simulink model "grid_afe_n"  (R2026a)
settings: Solver=ode23tb  StopTime=simlength  FixedStep=tc  MaxStep=glb_time.tc
values from neighbouring files (symbols this model uses):
  afe_ctrl = ctrl_afe_setup(glb_time.ts_afe, grid_emu.omega_grid_nom)    [init_model.m]
  afe_pwm_phase_shift_mod1 = 0    [init_model.m]
  afe_pwm_phase_shift_mod2 = 0    [init_model.m]
  afe_pwm_phase_shift_mod3 = 0    [init_model.m]
  afe_pwm_phase_shift_mod4 = 0    [init_model.m]
  filters = setup_global_filters(glb_time.ts_afe, glb_time.ts_inv, glb_time.ts_dab, glb_time.tc)    [init_model.m]
  frt_data = frt_settings(test_index, test_subindex, asymmetric_error_type,      enable_frt_1, enable_frt_2, start_time_LVRT, deepPOSxi, deepPOSeta, deepNEGxi, deepNEGeta)    [init_model.m]
  glb_time = timing_setup(fpwm_afe, trgo_afe, fpwm_inv, trgo_inv, fpwm_single_phase_inv, trgo_single_phase_inv, fpwm_dab, trgo_dab,      fpwm_psfbc, trgo_psfbc, fpwm_isop_rail, trgo_isop_rail, fpwm_cllc, trgo_cllc, t_measure, tc_factor, tc_decimation, delay_pwm, dead_time_afe,      dead_time_inv, dead_time_single_phase_inv, dead_time_dab, dead_time_psfbc, dead_time_isop_rail, dead_time_cllc)    [init_model.m]
  grid_emu = grid_three_phase_emulator('Dyn11', delta_star, grid_nominal_power, application_voltage, us1, us2, fgrid,                  eq_grid_inductance, eq_grid_resistance, eta, ucc, i1m, p_iron, n1, n2, core_area, core_length, mur,                  up_xi_pu_ref, up_eta_pu_ref, un_xi_pu_ref, un_eta_pu_ref)    [init_model.m]
  i_react_pos_ref_2 = -ixi_ref_mod1*tan(acos(0.95))    [init_model.m]
  i_react_pos_ref_3 = ixi_ref_mod1*tan(acos(0.95))    [init_model.m]
  ixi_ref_mod1 = -0.85    [init_model.m]
  ixi_ref_mod2 = -0.85    [init_model.m]
  ixi_ref_mod3 = -0.85    [init_model.m]
  ixi_ref_mod4 = -0.85    [init_model.m]
  ki_align = 18    [init_model.m]
  kp_align = 0.25    [init_model.m]
  lim_down_align = -0.05    [init_model.m]
  lim_up_align = 0.05    [init_model.m]
  mavarage_filter_frequency_base_order = 2    [init_model.m]
  time_gain_afe_module_1 = 1.0002    [init_model.m]
  time_gain_afe_module_2 = 1.0015    [init_model.m]
  time_gain_afe_module_3 = 0.9988    [init_model.m]
  time_gain_afe_module_4 = 1.0020    (= 1.002)    [init_model.m]
  time_i_react_pos_ref_1 = start_time_LVRT + error_length + 0.335    [init_model.m]
  time_i_react_pos_ref_2 = time_i_react_pos_ref_1 + 0.5    (= 0.5)    [init_model.m]
  u_cm_comp_mod1 = 0    [init_model.m]
  u_cm_comp_mod2 = -1    [init_model.m]
  u_cm_comp_mod3 = -1    [init_model.m]
  u_cm_comp_mod4 = -1    [init_model.m]
undefined symbols (not defined in the file or in its folder): hwdata, magnitude
libraries: fl_lib x113, nesl_utility x75, moving_average_filter x40, moving_average_filter_cc x32, sl_discontinuities x12, linear_double_integrator_observer_ccaller x8, discrete_time_low_pass_filter x4, threephase_inductor_lib x4, dclink_for_two_levels x4, three_phase_pwm_modulator x4, three_phase_inverter_ideal_switch_based_model x4, three_phase_inverter_igbt_advanced_thermal_model x4
(part 11 of 19)

== system grid_afe_n/afe_abc_mod1/AFE_control/afe_control/grid_voltage_phase_lock_loops/dq_pll/pll_stageB ==
  u_grid_pos_xi : Inport
  u_grid_pos_eta : Inport  Port=2
  -2<x<2 : Saturate  UpperLimit=2  LowerLimit=-2
  Constant4 : Constant  Value=grid_emu.omega_grid_nom
  Gain : Gain  Gain=1/grid_emu.omega_grid_nom
  Product1 : Product  RndMeth=Zero
  Product2 : Product  RndMeth=Zero
  Sum3 : Sum  SaturateOnIntegerOverflow=on
  Sum4 : Sum  SaturateOnIntegerOverflow=on
  Sum5 : Sum  Inputs=++|
  Terminator : Terminator
  Unit Delay1 : UnitDelay  SampleTime=-1
  Unit Delay2 : UnitDelay  SampleTime=-1
  Unit Delay4 : UnitDelay  SampleTime=-1
  bounder1 : MATLAB Function  TreatAsAtomicUnit=on
  double_integrator_observer : Subsystem
  kp : Gain  Gain=afe_ctrl.pll_i1*glb_time.ts_afe  SaturateOnIntegerOverflow=on  OutDataTypeStr=Inherit: Same as input  ParamDataTypeStr=Inherit: Same as input
  kp2 : Gain  Gain=glb_time.ts_afe  SaturateOnIntegerOverflow=on  OutDataTypeStr=Inherit: Same as input  ParamDataTypeStr=Inherit: Same as input
  scheduled-p-gain : Subsystem
      settings: PortSchema="{\"entries\":[{\"content\":{\"sides\":[{\"content\":{},\"type\":\"ConnectorPlacement.EquallySpacedRectSide\",\"uuid\":\"88e64df2-a299-4c1b-9bac-7a615cd04a00\"},{\"content\":{\"side\":\"RIGHT\"},\"type\":\"ConnectorPlacement.EquallySpacedRectSide\",\"uuid\":\"ef1d7318-b0e2-4e96-bf99-c42bb4ec5202\"},{\"content\":{\"connectorIds\":[\"In1\"],\"side\":\"TOP\"},\"type\":\"ConnectorPlacement.EquallySpacedRectSide\",\"uuid\":\"96582c59-f6c8-40f1-b3cf-394cc239c4b2\"},{\"content\":{\"connectorIds\":[\"Out1\"],\"side\":\"BOTTOM\"},\"type\":\"ConnectorPlacement.EquallySpacedRectSide\",\"uuid\":\"9ac5cd0d-958f-4b67-b4ea-90856a0aa038\"}]},\"type\":\"ConnectorPlacement.EquallySpacedConnector\",\"uuid\":\"ca37db80-6b94-4315-bd9c-66307567cd1f\"}],\"packageUris\":[\"http://schema.mathworks.com/mf0/Connector/R2020b\"],\"version\":\"1.0\"}"
  phase_grid_pll : Outport  VectorParamsAs1DForOutWhenUnconnected=off
  omega_grid_pu_pll : Outport  Port=2  VectorParamsAs1DForOutWhenUnconnected=off
  wires:
  Unit Delay4/1 -> Sum3/2
  Sum3/1 -> -2<x<2/1
  Sum4/1 -> bounder1/1(u)
  Unit Delay1/1 -> Sum4/2
  -2<x<2/1 -> Sum5/2, Unit Delay4/1  "i1"
  kp2/1 -> Sum4/1
  Constant4/1 -> Product2/2
  [Vgrid_unorm_dqpll] -> Product1/2
  kp/1 -> Sum3/1
  Sum5/1 -> Product2/1
  bounder1/1(y) -> Unit Delay1/1, Unit Delay2/1
  u_grid_pos_eta/1 -> Product1/1
  Product2/1 -> kp2/1
  Product1/1 -> scheduled-p-gain/1(In1), kp/1
  scheduled-p-gain/1(Out2) -> Sum5/1
  Unit Delay2/1 -> double_integrator_observer/1(phase), phase_grid_pll/1
  double_integrator_observer/1(omega_hat) -> Gain/1
  Gain/1 -> omega_grid_pu_pll/1
  u_grid_pos_xi/1 -> Terminator/1

== system grid_afe_n/afe_abc_mod1/AFE_control/afe_control/grid_voltage_phase_lock_loops/dq_pll_ccaller/first_harmonic_tracker_phase_u ==
  u : Inport
  Bus Selector : BusSelector  OutputSignals=output_pu_hat
  C Caller : CCaller  FunctionName=first_harmonic_tracker_process_simulink  PortSpecificationStruct="%)30     .    B \\   8    (     @         %    \"     D    !     0         %  0 \"0    $    _    07)G3F%M90  4&]R=$YA;64 4V-O<&4     26YD97@     5'EP90      4VEZ90      27-';&]B86P   X    P    !@    @    $          4    (     0    ,    !         !   P!O=70 #@   #     &    \"     0         !0    @    !     P    $         $  # &]U=  .    .     8    (    !          %    \"     $    &     0         0  ...(+4988 chars)"
  Constant : Constant  Value=glb_time.ts_afe
  Constant1 : Constant  Value=0
  Constant4 : Constant  Value=afe_ctrl.fht_grid.omega_fht
  Constant5 : Constant  Value=afe_ctrl.fht_grid.delta_fht
  Constant6 : Constant  Value=afe_ctrl.fht_grid.Ld_fht(1)
  Constant7 : Constant  Value=afe_ctrl.fht_grid.Ld_fht(2)
  Data Type Conversion{1..2,6..9} (6 alike) : DataTypeConversion  OutDataTypeStr=single  SaturateOnIntegerOverflow=off  RndMeth=Floor
  Data Type Conversion3 : DataTypeConversion  OutDataTypeStr=uint8  SaturateOnIntegerOverflow=off  RndMeth=Floor
  Data Type Conversion4 : DataTypeConversion  OutDataTypeStr=double  SaturateOnIntegerOverflow=off  RndMeth=Floor
  Data Type Conversion5 : DataTypeConversion  OutDataTypeStr=uint8  SaturateOnIntegerOverflow=off  RndMeth=Floor
  Step : Step  Time=0.0125  InitialValue=1  FinalValue=0
  u_hat : Outport
  wires:
  Data Type Conversion4/1 -> u_hat/1
  Data Type Conversion3/1 -> C Caller/1
  Data Type Conversion1/1 -> C Caller/3
  Data Type Conversion2/1 -> C Caller/2
  C Caller/1 -> Bus Selector/1
  Bus Selector/1 -> Data Type Conversion4/1  "<output_pu_hat>"
  Step/1 -> Data Type Conversion3/1
  u/1 -> Data Type Conversion2/1
  Constant/1 -> Data Type Conversion1/1
  Constant1/1 -> Data Type Conversion5/1
  Constant4/1 -> Data Type Conversion6/1
  Constant6/1 -> Data Type Conversion8/1
  Constant7/1 -> Data Type Conversion9/1
  Constant5/1 -> Data Type Conversion7/1
  Data Type Conversion5/1 -> C Caller/8
  Data Type Conversion6/1 -> C Caller/4
  Data Type Conversion7/1 -> C Caller/5
  Data Type Conversion8/1 -> C Caller/6
  Data Type Conversion9/1 -> C Caller/7

== system grid_afe_n/afe_abc_mod1/AFE_control/afe_control/grid_voltage_phase_lock_loops/dq_pll_ccaller/first_harmonic_tracker_phase_v ==
  u : Inport
  Bus Selector : BusSelector  OutputSignals=output_pu_hat
  C Caller : CCaller  FunctionName=first_harmonic_tracker_process_simulink  PortSpecificationStruct="%)30     .    B \\   8    (     @         %    \"     D    !     0         %  0 \"0    $    _    07)G3F%M90  4&]R=$YA;64 4V-O<&4     26YD97@     5'EP90      4VEZ90      27-';&]B86P   X    P    !@    @    $          4    (     0    ,    !         !   P!O=70 #@   #     &    \"     0         !0    @    !     P    $         $  # &]U=  .    .     8    (    !          %    \"     $    &     0         0  ...(+4988 chars)"
  Constant : Constant  Value=glb_time.ts_afe
  Constant1 : Constant  Value=2
  Constant4 : Constant  Value=afe_ctrl.fht_grid.omega_fht
  Constant5 : Constant  Value=afe_ctrl.fht_grid.delta_fht
  Constant6 : Constant  Value=afe_ctrl.fht_grid.Ld_fht(1)
  Constant7 : Constant  Value=afe_ctrl.fht_grid.Ld_fht(2)
  Data Type Conversion{1..2,6..9} (6 alike) : DataTypeConversion  OutDataTypeStr=single  SaturateOnIntegerOverflow=off  RndMeth=Floor
  Data Type Conversion3 : DataTypeConversion  OutDataTypeStr=uint8  SaturateOnIntegerOverflow=off  RndMeth=Floor
  Data Type Conversion4 : DataTypeConversion  OutDataTypeStr=double  SaturateOnIntegerOverflow=off  RndMeth=Floor
  Data Type Conversion5 : DataTypeConversion  OutDataTypeStr=uint8  SaturateOnIntegerOverflow=off  RndMeth=Floor
  Step : Step  Time=0.0125  InitialValue=1  FinalValue=0
  u_hat : Outport
  wires:
  Data Type Conversion9/1 -> C Caller/7
  Data Type Conversion8/1 -> C Caller/6
  Data Type Conversion7/1 -> C Caller/5
  Data Type Conversion6/1 -> C Caller/4
  Data Type Conversion5/1 -> C Caller/8
  Constant5/1 -> Data Type Conversion7/1
  Constant7/1 -> Data Type Conversion9/1
  Constant6/1 -> Data Type Conversion8/1
  Constant4/1 -> Data Type Conversion6/1
  Constant1/1 -> Data Type Conversion5/1
  Constant/1 -> Data Type Conversion1/1
  u/1 -> Data Type Conversion2/1
  Step/1 -> Data Type Conversion3/1
  Bus Selector/1 -> Data Type Conversion4/1  "<output_pu_hat>"
  C Caller/1 -> Bus Selector/1
  Data Type Conversion2/1 -> C Caller/2
  Data Type Conversion1/1 -> C Caller/3
  Data Type Conversion3/1 -> C Caller/1
  Data Type Conversion4/1 -> u_hat/1

== system grid_afe_n/afe_abc_mod1/AFE_control/afe_control/grid_voltage_phase_lock_loops/dq_pll_ccaller/first_harmonic_tracker_phase_w ==
  u : Inport
  Bus Selector : BusSelector  OutputSignals=output_pu_hat
  C Caller : CCaller  FunctionName=first_harmonic_tracker_process_simulink  PortSpecificationStruct="%)30     .    B \\   8    (     @         %    \"     D    !     0         %  0 \"0    $    _    07)G3F%M90  4&]R=$YA;64 4V-O<&4     26YD97@     5'EP90      4VEZ90      27-';&]B86P   X    P    !@    @    $          4    (     0    ,    !         !   P!O=70 #@   #     &    \"     0         !0    @    !     P    $         $  # &]U=  .    .     8    (    !          %    \"     $    &     0         0  ...(+4988 chars)"
  Constant : Constant  Value=glb_time.ts_afe
  Constant1 : Constant  Value=4
  Constant4 : Constant  Value=afe_ctrl.fht_grid.omega_fht
  Constant5 : Constant  Value=afe_ctrl.fht_grid.delta_fht
  Constant6 : Constant  Value=afe_ctrl.fht_grid.Ld_fht(1)
  Constant7 : Constant  Value=afe_ctrl.fht_grid.Ld_fht(2)
  Data Type Conversion{1..2,6..9} (6 alike) : DataTypeConversion  OutDataTypeStr=single  SaturateOnIntegerOverflow=off  RndMeth=Floor
  Data Type Conversion3 : DataTypeConversion  OutDataTypeStr=uint8  SaturateOnIntegerOverflow=off  RndMeth=Floor
  Data Type Conversion4 : DataTypeConversion  OutDataTypeStr=double  SaturateOnIntegerOverflow=off  RndMeth=Floor
  Data Type Conversion5 : DataTypeConversion  OutDataTypeStr=uint8  SaturateOnIntegerOverflow=off  RndMeth=Floor
  Step : Step  Time=0.0125  InitialValue=1  FinalValue=0
  u_hat : Outport
  wires:
  Data Type Conversion4/1 -> u_hat/1
  Data Type Conversion3/1 -> C Caller/1
  Data Type Conversion1/1 -> C Caller/3
  Data Type Conversion2/1 -> C Caller/2
  C Caller/1 -> Bus Selector/1
  Bus Selector/1 -> Data Type Conversion4/1  "<output_pu_hat>"
  Step/1 -> Data Type Conversion3/1
  u/1 -> Data Type Conversion2/1
  Constant/1 -> Data Type Conversion1/1
  Constant1/1 -> Data Type Conversion5/1
  Constant4/1 -> Data Type Conversion6/1
  Constant6/1 -> Data Type Conversion8/1
  Constant7/1 -> Data Type Conversion9/1
  Constant5/1 -> Data Type Conversion7/1
  Data Type Conversion5/1 -> C Caller/8
  Data Type Conversion6/1 -> C Caller/4
  Data Type Conversion7/1 -> C Caller/5
  Data Type Conversion8/1 -> C Caller/6
  Data Type Conversion9/1 -> C Caller/7

== system grid_afe_n/afe_abc_mod1/AFE_control/afe_control/grid_voltage_sequences/voltage_sequence_avg/average_filter ==
  v_grid_pos_xi : Inport
  v_grid_pos_eta : Inport  Port=2
  v_grid_neg_xi : Inport  Port=3
  v_grid_neg_eta : Inport  Port=4
  Abs : Abs  SaturateOnIntegerOverflow=off
  Gain : Gain  Gain=grid_emu.omega_grid_nom*mavarage_filter_frequency_base_order
  Saturation : Saturate  UpperLimit=2  LowerLimit=0.1
  dmavg_flt{,1..3} (4 alike) : moving_average_filter/dmavg_flt  ts=glb_time.ts_afe  enable_time=dmavg_filter_enable_time
  v_grid_pos_xi_avg : Outport
  v_grid_pos_eta_avg : Outport  Port=2
  v_grid_neg_xi_avg : Outport  Port=3
  v_grid_neg_eta_avg : Outport  Port=4
  wires:
  v_grid_neg_eta/1 -> dmavg_flt3/1
  v_grid_neg_xi/1 -> dmavg_flt2/1
  v_grid_pos_eta/1 -> dmavg_flt1/1
  dmavg_flt3/1 -> v_grid_neg_eta_avg/1
  dmavg_flt2/1 -> v_grid_neg_xi_avg/1
  dmavg_flt1/1 -> v_grid_pos_eta_avg/1
  Gain/1 -> dmavg_flt/2, dmavg_flt1/2, dmavg_flt2/2, dmavg_flt3/2
  dmavg_flt/1 -> v_grid_pos_xi_avg/1
  v_grid_pos_xi/1 -> dmavg_flt/1
  Abs/1 -> Saturation/1
  [omega_grid_pll_pu] -> Abs/1
  Saturation/1 -> Gain/1

== system grid_afe_n/afe_abc_mod1/AFE_control/afe_control/grid_voltage_sequences/voltage_sequence_avg/average_filter_ccaller ==
  v_grid_pos_xi : Inport
  v_grid_pos_eta : Inport  Port=2
  v_grid_neg_xi : Inport  Port=3
  v_grid_neg_eta : Inport  Port=4
  Abs : Abs  SaturateOnIntegerOverflow=off
  Gain : Gain  Gain=grid_emu.omega_grid_nom*mavarage_filter_frequency_base_order
  Saturation : Saturate  UpperLimit=2  LowerLimit=0.1
  dmavg_flt : moving_average_filter_cc/dmavg_flt  instance=0  ts=glb_time.ts_afe  enable_time=dmavg_filter_enable_time
  dmavg_flt1 : moving_average_filter_cc/dmavg_flt  instance=1  ts=glb_time.ts_afe  enable_time=dmavg_filter_enable_time
  dmavg_flt2 : moving_average_filter_cc/dmavg_flt  instance=2  ts=glb_time.ts_afe  enable_time=dmavg_filter_enable_time
  dmavg_flt3 : moving_average_filter_cc/dmavg_flt  instance=3  ts=glb_time.ts_afe  enable_time=dmavg_filter_enable_time
  v_grid_pos_xi_avg : Outport
  v_grid_pos_eta_avg : Outport  Port=2
  v_grid_neg_xi_avg : Outport  Port=3
  v_grid_neg_eta_avg : Outport  Port=4
  wires:
  v_grid_pos_xi/1 -> dmavg_flt/1
  dmavg_flt/1 -> v_grid_pos_xi_avg/1
  dmavg_flt1/1 -> v_grid_pos_eta_avg/1
  dmavg_flt2/1 -> v_grid_neg_xi_avg/1
  dmavg_flt3/1 -> v_grid_neg_eta_avg/1
  v_grid_pos_eta/1 -> dmavg_flt1/1
  v_grid_neg_xi/1 -> dmavg_flt2/1
  v_grid_neg_eta/1 -> dmavg_flt3/1
  Abs/1 -> Saturation/1
  Saturation/1 -> Gain/1
  [omega_grid_pll_pu] -> Abs/1
  Gain/1 -> dmavg_flt/2, dmavg_flt1/2, dmavg_flt3/2, dmavg_flt2/2

== system grid_afe_n/afe_abc_mod1/AFE_control/afe_control/phase_compensation_1/alignment_eval_afe1/pi ==
  u_ref : Inport
  u : Inport  Port=2
  1/Ti : Gain  Gain=kp  SaturateOnIntegerOverflow=on  OutDataTypeStr=Inherit: Same as input  ParamDataTypeStr=Inherit: Same as input
  Saturation : Saturate  UpperLimit=lim_up  LowerLimit=lim_down
  Sum1 : Sum  Inputs=+++  SaturateOnIntegerOverflow=on
  Sum2 : Sum  Inputs=-+  SaturateOnIntegerOverflow=on
  Sum3 : Sum  Inputs=-+  SaturateOnIntegerOverflow=on
  Unit Delay4 : UnitDelay  SampleTime=-1
  kp : Gain  Gain=ki  SaturateOnIntegerOverflow=on  OutDataTypeStr=Inherit: Same as input  ParamDataTypeStr=Inherit: Same as input
  y : Outport
  wires:
  1/Ti/1 -> Sum1/1, Sum3/1
  kp/1 -> Sum1/2
  Sum3/1 -> Unit Delay4/1
  Unit Delay4/1 -> Sum1/3
  u_ref/1 -> Sum2/2
  u/1 -> Sum2/1
  Sum2/1 -> kp/1, 1/Ti/1
  Sum1/1 -> Saturation/1
  Saturation/1 -> Sum3/2, y/1

== system grid_afe_n/afe_abc_mod2/AFE_control/afe_control/FRT-VDE4110/FRT-Detection/voltage_rate_measure_neg ==
  v_grid_neg_xi_avg : Inport
  Abs1 : Abs  SaturateOnIntegerOverflow=off
  Terminator : Terminator
  linear_double_integrator_observer_ccaller : linear_double_integrator_observer_ccaller/linear_double_integrator_observer_ccaller  kx_m=afe_ctrl.vr_obs.kx  kv_m=afe_ctrl.vr_obs.kv  ts_m=glb_time.ts_afe  time_release=0.025  instance=2  tc_m=-1
  vxi_neg_dot : Outport
  wires:
  Abs1/1 -> vxi_neg_dot/1  "vxi_neg_dot"
  v_grid_neg_xi_avg/1 -> linear_double_integrator_observer_ccaller/1
  linear_double_integrator_observer_ccaller/2 -> Abs1/1
  linear_double_integrator_observer_ccaller/1 -> Terminator/1  "x_hat_ccaller"

== system grid_afe_n/afe_abc_mod2/AFE_control/afe_control/FRT-VDE4110/FRT-Detection/voltage_rate_measure_pos ==
  v_grid_pos_xi_avg : Inport
  Abs : Abs  SaturateOnIntegerOverflow=off
  Terminator : Terminator
  linear_double_integrator_observer_ccaller : linear_double_integrator_observer_ccaller/linear_double_integrator_observer_ccaller  kx_m=afe_ctrl.vr_obs.kx  kv_m=afe_ctrl.vr_obs.kv  ts_m=glb_time.ts_afe  time_release=0.025  instance=0  tc_m=-1
  vxi_pos_dot : Outport
  wires:
  v_grid_pos_xi_avg/1 -> linear_double_integrator_observer_ccaller/1
  Abs/1 -> vxi_pos_dot/1  "vxi_pos_dot"
  linear_double_integrator_observer_ccaller/2 -> Abs/1
  linear_double_integrator_observer_ccaller/1 -> Terminator/1  "x_hat_ccaller"

== system grid_afe_n/afe_abc_mod2/AFE_control/afe_control/FRT-VDE4110/FRT-PosNegReactiveCurrentReferences/avg_flt_500ms ==
  In1 : Inport
  Constant : Constant  Value=2*pi/500e-3
  Constant1 : Constant  Value=glb_time.ts_afe
  Constant2 : Constant
  Sum : Sum  Inputs=|-+
  avg_flt_1 : MATLAB Function  TreatAsAtomicUnit=on
  Out1 : Outport  VectorParamsAs1DForOutWhenUnconnected=off
  wires:
  Sum/1 -> avg_flt_1/4(enable)
  [frt_active] -> Sum/1
  Constant2/1 -> Sum/2
  In1/1 -> avg_flt_1/1(x)  "input"
  Constant/1 -> avg_flt_1/2(w)
  Constant1/1 -> avg_flt_1/3(ts)
  avg_flt_1/1(y1) -> Out1/1  "output"

== system grid_afe_n/afe_abc_mod2/AFE_control/afe_control/FRT-VDE4110/FRT-PosNegReactiveCurrentReferences/avg_flt_500ms1 ==
  In1 : Inport
  Constant : Constant  Value=2*pi/500e-3
  Constant1 : Constant  Value=glb_time.ts_afe
  Constant2 : Constant
  Sum : Sum  Inputs=|-+
  avg_flt_1 : MATLAB Function  TreatAsAtomicUnit=on
  Out1 : Outport  VectorParamsAs1DForOutWhenUnconnected=off
  wires:
  avg_flt_1/1(y1) -> Out1/1  "output"
  Constant1/1 -> avg_flt_1/3(ts)
  Constant/1 -> avg_flt_1/2(w)
  In1/1 -> avg_flt_1/1(x)  "input"
  Constant2/1 -> Sum/2
  [frt_active] -> Sum/1
  Sum/1 -> avg_flt_1/4(enable)

== system grid_afe_n/afe_abc_mod2/AFE_control/afe_control/FRT-VDE4110/FRT-PosNegReactiveCurrentReferences/avg_flt_500ms2 ==
  In1 : Inport
  Constant : Constant  Value=2*pi/500e-3
  Constant1 : Constant  Value=glb_time.ts_afe
  Constant2 : Constant
  Sum : Sum  Inputs=|-+
  avg_flt_1 : MATLAB Function  TreatAsAtomicUnit=on
  Out1 : Outport  VectorParamsAs1DForOutWhenUnconnected=off
  wires:
  Sum/1 -> avg_flt_1/4(enable)
  [frt_active] -> Sum/1
  Constant2/1 -> Sum/2
  In1/1 -> avg_flt_1/1(x)  "input"
  Constant/1 -> avg_flt_1/2(w)
  Constant1/1 -> avg_flt_1/3(ts)
  avg_flt_1/1(y1) -> Out1/1  "output"

== system grid_afe_n/afe_abc_mod2/AFE_control/afe_control/FRT-VDE4110/FRT-PosNegReactiveCurrentReferences/avg_flt_500ms3 ==
  In1 : Inport
  Constant : Constant  Value=2*pi/500e-3
  Constant1 : Constant  Value=glb_time.ts_afe
  Constant2 : Constant
  Sum : Sum  Inputs=|-+
  avg_flt_1 : MATLAB Function  TreatAsAtomicUnit=on
  Out1 : Outport  VectorParamsAs1DForOutWhenUnconnected=off
  wires:
  avg_flt_1/1(y1) -> Out1/1  "output"
  Constant1/1 -> avg_flt_1/3(ts)
  Constant/1 -> avg_flt_1/2(w)
  In1/1 -> avg_flt_1/1(x)  "input"
  Constant2/1 -> Sum/2
  [frt_active] -> Sum/1
  Sum/1 -> avg_flt_1/4(enable)

== system grid_afe_n/afe_abc_mod2/AFE_control/afe_control/FRT-VDE4110/FRT-PosNegReactiveCurrentReferences/positive_reactive_current_reference ==
  Step : Step  Time=time_i_react_pos_ref_1  InitialValue=i_react_pos_ref_1  FinalValue=i_react_pos_ref_2
  Step1 : Step  Time=time_i_react_pos_ref_2  FinalValue=i_react_pos_ref_3-i_react_pos_ref_2
  Sum7 : Sum  Inputs=|++
  i_react_pos_ref : Outport
  wires:
  Sum7/1 -> i_react_pos_ref/1
  Step1/1 -> Sum7/2
  Step/1 -> Sum7/1

== system grid_afe_n/afe_abc_mod2/AFE_control/afe_control/FRT-VDE4110/FRT-PosNegReactiveCurrentReferences/u_161Hz_flt1 ==
  input : Inport
  Gain3 : Gain  Gain=filters.afe.g1_161Hz
  Gain6 : Gain  Gain=filters.afe.g0_161Hz
  Sum : Sum  Inputs=|++
  Unit Delay1 : UnitDelay  SampleTime=-1
  output : Outport  VectorParamsAs1DForOutWhenUnconnected=off
  wires:
  Sum/1 -> output/1, Unit Delay1/1
  Gain3/1 -> Sum/2
  Unit Delay1/1 -> Gain3/1
  input/1 -> Gain6/1
  Gain6/1 -> Sum/1

== system grid_afe_n/afe_abc_mod2/AFE_control/afe_control/FRT-VDE4110/FRT-PosNegReactiveCurrentReferences/u_161Hz_flt2 ==
  input : Inport
  Gain3 : Gain  Gain=filters.afe.g1_161Hz
  Gain6 : Gain  Gain=filters.afe.g0_161Hz
  Sum : Sum  Inputs=|++
  Unit Delay1 : UnitDelay  SampleTime=-1
  output : Outport  VectorParamsAs1DForOutWhenUnconnected=off
  wires:
  Gain6/1 -> Sum/1
  input/1 -> Gain6/1
  Unit Delay1/1 -> Gain3/1
  Gain3/1 -> Sum/2
  Sum/1 -> Unit Delay1/1, output/1

== system grid_afe_n/afe_abc_mod2/AFE_control/afe_control/FRT-VDE4110/FRT-PosNegReactiveCurrentReferences/u_161Hz_flt3 ==
  input : Inport
  Gain3 : Gain  Gain=filters.afe.g1_161Hz
  Gain6 : Gain  Gain=filters.afe.g0_161Hz
  Sum : Sum  Inputs=|++
  Unit Delay1 : UnitDelay  SampleTime=-1
  output : Outport  VectorParamsAs1DForOutWhenUnconnected=off
  wires:
  Sum/1 -> output/1, Unit Delay1/1
  Gain3/1 -> Sum/2
  Unit Delay1/1 -> Gain3/1
  input/1 -> Gain6/1
  Gain6/1 -> Sum/1

== system grid_afe_n/afe_abc_mod2/AFE_control/afe_control/current_ctrl/inner_current_ctrl/rpi_phase_a ==
  In1 : Inport
  In2 : Inport  Port=2
  Add : Sum
  Cresd : Gain  Gain=afe_ctrl.res_pi.Cresd  Multiplication=Matrix(K*u)
  Gain : Gain  Gain=afe_ctrl.res_pi.kp_rpi
  Gain1 : Gain  Gain=afe_ctrl.res_pi.ki_rpi
  Gain2 : Gain  Gain=afe_ctrl.res_pi.Bresd  Multiplication=Matrix(K*u)
  Gain3 : Gain  Gain=afe_ctrl.res_pi.Aresd  Multiplication=Matrix(K*u)
  Sum : Sum  Inputs=|+-
  Sum2 : Sum  Inputs=|++  SaturateOnIntegerOverflow=on
  Unit Delay : UnitDelay  InitialCondition=[0 0]  SampleTime=-1
  Out1 : Outport
  wires:
  Cresd/1 -> Add/2  "y(k)"
  Gain3/1 -> Sum2/2
  Sum2/1 -> Unit Delay/1  "x(k+1)"
  Unit Delay/1 -> Cresd/1, Gain3/1  "x(k)"
  Gain2/1 -> Sum2/1
  Gain1/1 -> Gain2/1  "u(k)"
  Gain/1 -> Add/1
  Sum/1 -> Gain/1, Gain1/1
  Add/1 -> Out1/1  "da"
  In2/1 -> Sum/2  "isa"
  In1/1 -> Sum/1  "isa_ref"

== system grid_afe_n/afe_abc_mod2/AFE_control/afe_control/current_ctrl/inner_current_ctrl/rpi_phase_b ==
  In1 : Inport
  In2 : Inport  Port=2
  Add : Sum
  Cresd : Gain  Gain=afe_ctrl.res_pi.Cresd  Multiplication=Matrix(K*u)
  Gain : Gain  Gain=afe_ctrl.res_pi.kp_rpi
  Gain1 : Gain  Gain=afe_ctrl.res_pi.ki_rpi
  Gain2 : Gain  Gain=afe_ctrl.res_pi.Bresd  Multiplication=Matrix(K*u)
  Gain3 : Gain  Gain=afe_ctrl.res_pi.Aresd  Multiplication=Matrix(K*u)
  Sum : Sum  Inputs=|+-
  Sum2 : Sum  Inputs=|++  SaturateOnIntegerOverflow=on
  Unit Delay : UnitDelay  InitialCondition=[0 0]  SampleTime=-1
  Out1 : Outport
  wires:
  In1/1 -> Sum/1  "isa_ref"
  In2/1 -> Sum/2  "isa"
  Add/1 -> Out1/1  "da"
  Sum/1 -> Gain1/1, Gain/1
  Gain/1 -> Add/1
  Gain1/1 -> Gain2/1  "u(k)"
  Gain2/1 -> Sum2/1
  Unit Delay/1 -> Gain3/1, Cresd/1  "x(k)"
  Sum2/1 -> Unit Delay/1  "x(k+1)"
  Gain3/1 -> Sum2/2
  Cresd/1 -> Add/2  "y(k)"

== system grid_afe_n/afe_abc_mod2/AFE_control/afe_control/current_ctrl/inner_current_ctrl/rpi_phase_c ==
  In1 : Inport
  In2 : Inport  Port=2
  Add : Sum
  Cresd : Gain  Gain=afe_ctrl.res_pi.Cresd  Multiplication=Matrix(K*u)
  Gain : Gain  Gain=afe_ctrl.res_pi.kp_rpi
  Gain1 : Gain  Gain=afe_ctrl.res_pi.ki_rpi
  Gain2 : Gain  Gain=afe_ctrl.res_pi.Bresd  Multiplication=Matrix(K*u)
  Gain3 : Gain  Gain=afe_ctrl.res_pi.Aresd  Multiplication=Matrix(K*u)
  Sum : Sum  Inputs=|+-
  Sum2 : Sum  Inputs=|++  SaturateOnIntegerOverflow=on
  Unit Delay : UnitDelay  InitialCondition=[0 0]  SampleTime=-1
  Out1 : Outport
  wires:
  Cresd/1 -> Add/2  "y(k)"
  Gain3/1 -> Sum2/2
  Sum2/1 -> Unit Delay/1  "x(k+1)"
  Unit Delay/1 -> Cresd/1, Gain3/1  "x(k)"
  Gain2/1 -> Sum2/1
  Gain1/1 -> Gain2/1  "u(k)"
  Gain/1 -> Add/1
  Sum/1 -> Gain/1, Gain1/1
  Add/1 -> Out1/1  "da"
  In2/1 -> Sum/2  "isa"
  In1/1 -> Sum/1  "isa_ref"

== system grid_afe_n/afe_abc_mod2/AFE_control/afe_control/current_ctrl/inner_current_ctrl/zero_current_ctrl ==
  d_abc : Inport
  Bus Creator1 : BusCreator  Inputs=3
  antiwind_up : Subsystem
  iz : Subsystem
  zero_sequence_current_ctrl : Subsystem
  u_ctrl_out : Outport
  wires:
  zero_sequence_current_ctrl/1(ugamma_afe) -> Bus Creator1/3  "ugamma_afe"
  iz/1(iz) -> zero_sequence_current_ctrl/1(iz)
  antiwind_up/2(ubeta_afe) -> Bus Creator1/2  "ubeta_afe"
  antiwind_up/1(ualpha_afe) -> Bus Creator1/1  "ualpha_afe"
  d_abc/1 -> antiwind_up/1(d_abc)  "d_abc"
  Bus Creator1/1 -> u_ctrl_out/1

== system grid_afe_n/afe_abc_mod2/AFE_control/afe_control/grid_current_sequences_and_reactive_pwr_ctrl/current_sequence_avg/average_filter ==
  i_grid_pos_xi : Inport
  i_grid_pos_eta : Inport  Port=2
  i_grid_neg_xi : Inport  Port=3
  i_grid_neg_eta : Inport  Port=4
  Abs : Abs  SaturateOnIntegerOverflow=off
  Gain : Gain  Gain=grid_emu.omega_grid_nom*mavarage_filter_frequency_base_order
  Saturation : Saturate  UpperLimit=2  LowerLimit=0.1
  dmavg_flt{,1..3} (4 alike) : moving_average_filter/dmavg_flt  ts=glb_time.ts_afe  enable_time=dmavg_filter_enable_time
  i_grid_pos_xi_avg : Outport
  i_grid_pos_eta_avg : Outport  Port=2
  i_grid_neg_xi_avg : Outport  Port=3
  i_grid_neg_eta_avg : Outport  Port=4
  wires:
  [omega_grid_pll_pu] -> Abs/1
  Saturation/1 -> Gain/1
  Abs/1 -> Saturation/1
  dmavg_flt1/1 -> i_grid_pos_eta_avg/1
  dmavg_flt3/1 -> i_grid_neg_eta_avg/1
  i_grid_neg_xi/1 -> dmavg_flt2/1
  dmavg_flt2/1 -> i_grid_neg_xi_avg/1
  i_grid_pos_xi/1 -> dmavg_flt/1
  i_grid_neg_eta/1 -> dmavg_flt3/1
  dmavg_flt/1 -> i_grid_pos_xi_avg/1
  Gain/1 -> dmavg_flt2/2, dmavg_flt3/2, dmavg_flt1/2, dmavg_flt/2
  i_grid_pos_eta/1 -> dmavg_flt1/1

== system grid_afe_n/afe_abc_mod2/AFE_control/afe_control/grid_current_sequences_and_reactive_pwr_ctrl/current_sequence_avg/average_filter_ccaller ==
  i_grid_pos_xi : Inport
  i_grid_pos_eta : Inport  Port=2
  i_grid_neg_xi : Inport  Port=3
  i_grid_neg_eta : Inport  Port=4
  Abs : Abs  SaturateOnIntegerOverflow=off
  Gain : Gain  Gain=grid_emu.omega_grid_nom*mavarage_filter_frequency_base_order
  Saturation : Saturate  UpperLimit=2  LowerLimit=0.1
  dmavg_flt : moving_average_filter_cc/dmavg_flt  instance=4  ts=glb_time.ts_afe  enable_time=dmavg_filter_enable_time
  dmavg_flt1 : moving_average_filter_cc/dmavg_flt  instance=5  ts=glb_time.ts_afe  enable_time=dmavg_filter_enable_time
  dmavg_flt2 : moving_average_filter_cc/dmavg_flt  instance=6  ts=glb_time.ts_afe  enable_time=dmavg_filter_enable_time
  dmavg_flt3 : moving_average_filter_cc/dmavg_flt  instance=7  ts=glb_time.ts_afe  enable_time=dmavg_filter_enable_time
  i_grid_pos_xi_avg : Outport
  i_grid_pos_eta_avg : Outport  Port=2
  i_grid_neg_xi_avg : Outport  Port=3
  i_grid_neg_eta_avg : Outport  Port=4
  wires:
  [omega_grid_pll_pu] -> Abs/1
  Saturation/1 -> Gain/1
  Abs/1 -> Saturation/1
  i_grid_pos_eta/1 -> dmavg_flt1/1
  Gain/1 -> dmavg_flt2/2, dmavg_flt3/2, dmavg_flt1/2, dmavg_flt/2
  dmavg_flt/1 -> i_grid_pos_xi_avg/1
  i_grid_neg_eta/1 -> dmavg_flt3/1
  i_grid_pos_xi/1 -> dmavg_flt/1
  dmavg_flt2/1 -> i_grid_neg_xi_avg/1
  i_grid_neg_xi/1 -> dmavg_flt2/1
  dmavg_flt3/1 -> i_grid_neg_eta_avg/1
  dmavg_flt1/1 -> i_grid_pos_eta_avg/1

== system grid_afe_n/afe_abc_mod2/AFE_control/afe_control/grid_current_sequences_and_reactive_pwr_ctrl/sequences_current_control/Negative-Seq. eta-Control ==
  ff : Inport
  e : Inport  Port=2
  1/Ti : Gain  Gain=afe_ctrl.kp_rc_neg_grid  SaturateOnIntegerOverflow=on  OutDataTypeStr=Inherit: Same as input  ParamDataTypeStr=Inherit: Same as input
  Saturation : Saturate  UpperLimit=afe_ctrl.ieta_neg_ref_lim  LowerLimit=-afe_ctrl.ieta_neg_ref_lim
  Sum : Sum  Inputs=|++
  Sum2 : Sum  Inputs=+++  SaturateOnIntegerOverflow=on
  Sum3 : Sum  Inputs=-+  SaturateOnIntegerOverflow=on
  Unit Delay4 : UnitDelay  SampleTime=-1
  kp : Gain  Gain=afe_ctrl.ki_rc_neg_grid*glb_time.ts_afe  SaturateOnIntegerOverflow=on  OutDataTypeStr=Inherit: Same as input  ParamDataTypeStr=Inherit: Same as input
  u : Outport  VectorParamsAs1DForOutWhenUnconnected=off
  wires:
  ff/1 -> Sum/2
  e/1 -> kp/1, 1/Ti/1  "e"
  Sum/1 -> u/1
  Saturation/1 -> Sum3/2, Sum/1
  1/Ti/1 -> Sum3/1, Sum2/1
  Sum2/1 -> Saturation/1
  kp/1 -> Sum2/2
  Sum3/1 -> Unit Delay4/1
  Unit Delay4/1 -> Sum2/3

== system grid_afe_n/afe_abc_mod2/AFE_control/afe_control/grid_current_sequences_and_reactive_pwr_ctrl/sequences_current_control/Negative-Seq. xi-Control ==
  ff : Inport
  e : Inport  Port=2
  1/Ti : Gain  Gain=afe_ctrl.kp_rc_neg_grid  SaturateOnIntegerOverflow=on  OutDataTypeStr=Inherit: Same as input  ParamDataTypeStr=Inherit: Same as input
  Saturation : Saturate  UpperLimit=afe_ctrl.ieta_pos_ref_lim  LowerLimit=-afe_ctrl.ieta_pos_ref_lim
  Sum : Sum  Inputs=|++
  Sum2 : Sum  Inputs=+++  SaturateOnIntegerOverflow=on
  Sum3 : Sum  Inputs=-+  SaturateOnIntegerOverflow=on
  Unit Delay4 : UnitDelay  SampleTime=-1
  kp : Gain  Gain=afe_ctrl.ki_rc_neg_grid*glb_time.ts_afe  SaturateOnIntegerOverflow=on  OutDataTypeStr=Inherit: Same as input  ParamDataTypeStr=Inherit: Same as input
  u : Outport  VectorParamsAs1DForOutWhenUnconnected=off
  wires:
  ff/1 -> Sum/2
  e/1 -> kp/1, 1/Ti/1  "e"
  Sum/1 -> u/1
  Saturation/1 -> Sum3/2, Sum/1
  1/Ti/1 -> Sum3/1, Sum2/1
  Sum2/1 -> Saturation/1
  kp/1 -> Sum2/2
  Sum3/1 -> Unit Delay4/1
  Unit Delay4/1 -> Sum2/3

== system grid_afe_n/afe_abc_mod2/AFE_control/afe_control/grid_current_sequences_and_reactive_pwr_ctrl/sequences_current_control/Positive-Seq. eta-Control ==
  ff : Inport
  e : Inport  Port=2
  1/Ti : Gain  Gain=afe_ctrl.kp_rc_pos_grid  SaturateOnIntegerOverflow=on  OutDataTypeStr=Inherit: Same as input  ParamDataTypeStr=Inherit: Same as input
  Saturation : Saturate  UpperLimit=afe_ctrl.ieta_pos_ref_lim  LowerLimit=-afe_ctrl.ieta_pos_ref_lim
  Sum : Sum  Inputs=|++
  Sum2 : Sum  Inputs=+++  SaturateOnIntegerOverflow=on
  Sum3 : Sum  Inputs=-+  SaturateOnIntegerOverflow=on
  Unit Delay4 : UnitDelay  SampleTime=-1
  kp : Gain  Gain=afe_ctrl.ki_rc_pos_grid*glb_time.ts_afe  SaturateOnIntegerOverflow=on  OutDataTypeStr=Inherit: Same as input  ParamDataTypeStr=Inherit: Same as input
  u : Outport  VectorParamsAs1DForOutWhenUnconnected=off
  wires:
  ff/1 -> Sum/2
  e/1 -> kp/1, 1/Ti/1  "e"
  Sum/1 -> u/1
  Saturation/1 -> Sum3/2, Sum/1
  1/Ti/1 -> Sum3/1, Sum2/1
  Sum2/1 -> Saturation/1
  kp/1 -> Sum2/2
  Sum3/1 -> Unit Delay4/1
  Unit Delay4/1 -> Sum2/3

== system grid_afe_n/afe_abc_mod2/AFE_control/afe_control/grid_voltage_phase_lock_loops/FHT-PLL/pll_stageA ==
  gamma_grid : Inport
  ug_abc_pu : Inport  Port=2
  Demux : Demux  Outputs=3
  Math Function : Math  Operator=magnitude^2  SignedPower=on
  Math Function1 : Math  Operator=magnitude^2  SignedPower=on
  Reciprocal Sqrt : Sqrt  Operator=rSqrt
  Saturation : Saturate  UpperLimit=inf  LowerLimit=0.02
  Sum : Sum  Inputs=|++
  filter_and_transformation : Subsystem
  sequences : Subsystem
  u_grid_xi : Outport  VectorParamsAs1DForOutWhenUnconnected=off
  u_grid_eta : Outport  Port=2  VectorParamsAs1DForOutWhenUnconnected=off
  tag scope: Vgrid_unorm_fht=scoped
  wires:
  Saturation/1 -> Reciprocal Sqrt/1
  Reciprocal Sqrt/1 -> [Vgrid_unorm_fht]
  Sum/1 -> Saturation/1
  Math Function1/1 -> Sum/2
  Math Function/1 -> Sum/1
  filter_and_transformation/2(ug_beta) -> sequences/2(u_grid_beta), Math Function1/1
  filter_and_transformation/1(ug_alpha) -> sequences/1(u_grid_alpha), Math Function/1
  Demux/3 -> filter_and_transformation/3(ug_c)
  Demux/2 -> filter_and_transformation/2(ug_b)
  Demux/1 -> filter_and_transformation/1(ug_a)
  ug_abc_pu/1 -> Demux/1
  sequences/1(u_grid_xi) -> u_grid_xi/1
  sequences/2(u_grid_eta) -> u_grid_eta/1
  gamma_grid/1 -> sequences/3(phase_angle)

== system grid_afe_n/afe_abc_mod2/AFE_control/afe_control/grid_voltage_phase_lock_loops/FHT-PLL/pll_stageB ==
  u_grid_pos_xi : Inport
  u_grid_pos_eta : Inport  Port=2
  Constant4 : Constant  Value=grid_emu.omega_grid_nom
  Gain : Gain  Gain=-1
  Product : Product  RndMeth=Zero
  Product1 : Product  RndMeth=Zero
  Product2 : Product  RndMeth=Zero
  Sum3 : Sum  SaturateOnIntegerOverflow=on
  Sum4 : Sum  SaturateOnIntegerOverflow=on
  Sum5 : Sum  Inputs=++|
  Terminator : Terminator
  Unit Delay1 : UnitDelay  SampleTime=-1
  Unit Delay2 : UnitDelay  SampleTime=-1
  Unit Delay4 : UnitDelay  SampleTime=-1
  bounder1 : MATLAB Function  TreatAsAtomicUnit=on
  double_integrator_observer : Subsystem
  kp : Gain  Gain=afe_ctrl.pll_i1_fht*glb_time.ts_afe  SaturateOnIntegerOverflow=on  OutDataTypeStr=Inherit: Same as input  ParamDataTypeStr=Inherit: Same as input
  kp1 : Gain  Gain=afe_ctrl.pll_p_fht  SaturateOnIntegerOverflow=on  OutDataTypeStr=Inherit: Same as input  ParamDataTypeStr=Inherit: Same as input
  kp2 : Gain  Gain=glb_time.ts_afe  SaturateOnIntegerOverflow=on  OutDataTypeStr=Inherit: Same as input  ParamDataTypeStr=Inherit: Same as input
  kp3 : Gain  Gain=1/grid_emu.omega_grid_nom  SaturateOnIntegerOverflow=on  OutDataTypeStr=Inherit: Same as input  ParamDataTypeStr=Inherit: Same as input
  gamma_grid_ddsrf_pll : Outport  VectorParamsAs1DForOutWhenUnconnected=off
  omega_grid_ddsrf_pll : Outport  Port=2  VectorParamsAs1DForOutWhenUnconnected=off
  wires:
  Unit Delay2/1 -> gamma_grid_ddsrf_pll/1, double_integrator_observer/1(theta)
  kp1/1 -> Sum5/1
  Product2/1 -> kp2/1
  u_grid_pos_eta/1 -> Product1/1
  u_grid_pos_xi/1 -> Product/1
  bounder1/1(y) -> Unit Delay1/1, Unit Delay2/1
  Sum5/1 -> Product2/1
  kp/1 -> Sum3/1
  [Vgrid_unorm_fht] -> Product1/2, Product/2
  Constant4/1 -> Product2/2
  kp2/1 -> Sum4/1
  Sum3/1 -> Unit Delay4/1, Sum5/2  "i1"
  Unit Delay1/1 -> Sum4/2
  Sum4/1 -> bounder1/1(u)
  Unit Delay4/1 -> Sum3/2
  double_integrator_observer/1(omega_hat) -> kp3/1
  Product/1 -> Terminator/1
  kp3/1 -> omega_grid_ddsrf_pll/1
  Product1/1 -> Gain/1
  Gain/1 -> kp1/1, kp/1
